simulink model "Buck"  (R2021b)
settings: Solver=VariableStepAuto  StartTime=0.0  StopTime=10.0  RelTol=1e-3
libraries: spsCurrentMeasurementLib x2, spsSeriesRLCBranchLib x2, spsDCVoltageSourceLib x1, spsDiodeLib x1, spsMosfetLib x1, spsVoltageMeasurementLib x1, spspowerguiLib x1
settings Model: Creator=szenia  LastModifiedBy=szenia

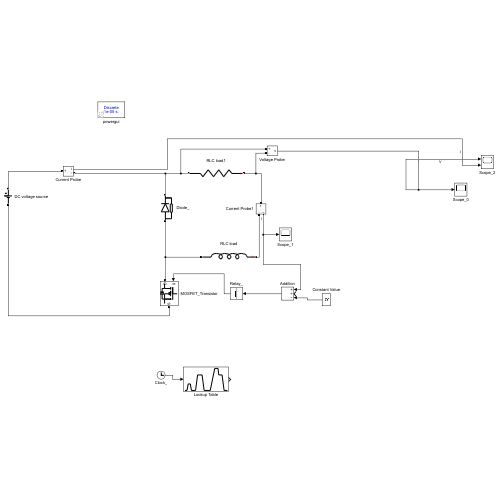
[thumbnail: Simulink's stored preview of the top-level diagram]
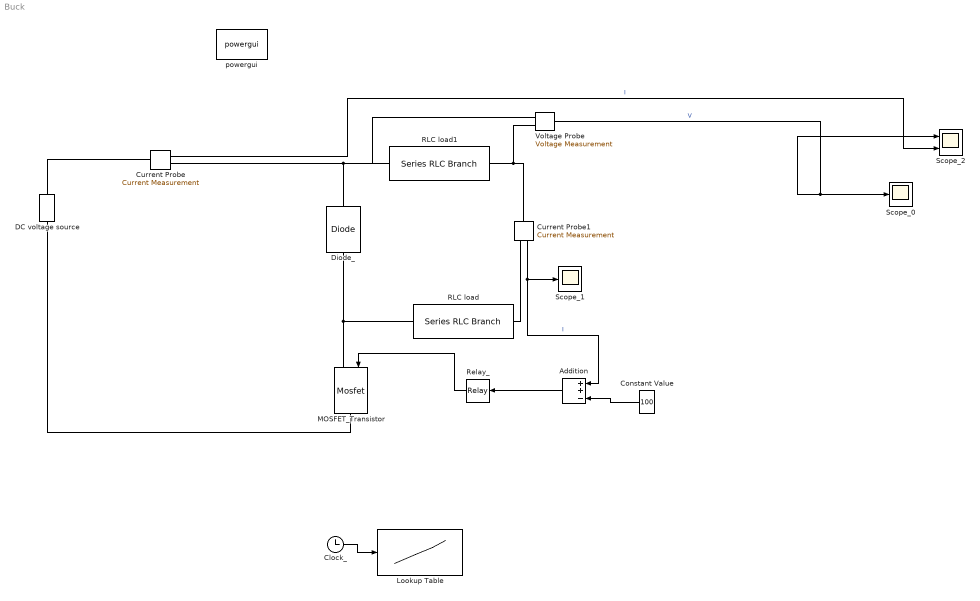
== system Buck ==
  Addition : Sum  Inputs=++-
  Clock_ : Clock
  Constant Value : Constant  Value=100
  Current Probe : spsCurrentMeasurementLib/Current Measurement  PhasorSimulation=off  OutputType=Complex  PSBequivalent=0
  Current Probe1 : spsCurrentMeasurementLib/Current Measurement  PhasorSimulation=off  OutputType=Complex  PSBequivalent=0
  DC voltage source : spsDCVoltageSourceLib/DC Voltage Source  Amplitude=250  Measurements=None
  Diode_ : spsDiodeLib/Diode  Ron=0.001  Lon=0  Vf=0.8  IC=0  UseSnubber=off  Rs=500  Cs=250e-9  Measurements=off
  Lookup Table : Lookup  InputValues=[0,10,15,25,30,50,60,80,90,120,140,155,160,175,185,200]  Table=[0,0,15,15,0,0,35,35,0,0,50,50,35,35,0,0]
  MOSFET_Transistor : spsMosfetLib/Mosfet  Ron=0.004  Lon=0  Rd=0.01  Vfd=0  IC=0  Rs=1e5  Cs=inf  Measurements=off
  RLC load : spsSeriesRLCBranchLib/Series RLC Branch  LConnTagsString=__new0  RConnTagsString=__new0  BranchType=L  Resistance=1  Inductance=10e-3  SetiL0=off  InitialCurrent=0  Capacitance=0  Setx0=off  InitialVoltage=0  Measurements=Branch current
  RLC load1 : spsSeriesRLCBranchLib/Series RLC Branch  LConnTagsString=__new0  RConnTagsString=__new0  BranchType=R  Resistance=1  Inductance=1e-2  SetiL0=off  InitialCurrent=0  Capacitance=0  Setx0=off  InitialVoltage=0  Measurements=Branch current
  Relay_ : Relay  OnSwitchValue=1  OffSwitchValue=-1  OnOutputValue=0  OffOutputValue=1
  Scope_0 : Scope
  Scope_1 : Scope
  Scope_2 : Scope  NumInputPorts=2
  Voltage Probe : spsVoltageMeasurementLib/Voltage Measurement  PhasorSimulation=off  OutputType=Complex  PSBequivalent=0
  powergui : spspowerguiLib/powergui  Priority=1  SimulationMode=Discrete  SampleTime=1e-5  frequency=60  Iterations=50  frequencyindice=0  Pbase=100e6  ErrMax=1e-4  UnitsV=kV  UnitsW=MW  buscounter=0  FunctionMessages=off  echomessages=off  EnableUseOfTLC=off  CurrentSourceSwitches=off  DisableSnubberDevices=off  DisableRonSwitches=off  DisableVfSwitches=off  DisplayEquations=off  AutomaticDiscreteSolvers=off  SolverType=Tustin/Backward Euler (TBE)  Interpol=off  ExternalGateDelay=off  methode=off  Ts=100  x0status=zero  SPID=on  SwTol=0  HookPort=off  NonlinearTolerance=1e-4  nMaxIteration=100  ContinueOnMaxIteration=off  RestoreLinks=warning  ResistiveCurrentMeasurement=off  Frange=[0:2:500]  Ylog=off  Xlog=on  ShowGrid=off  save=off  variable=ZData  structure=0  ZoomFFT=off  StartTime=0.0  cycles=1  DisplayStyle=1  fundamental=60  FreqAxis=off  MaxFrequency=1000  frequencyindicesteady=1  RmsSteady=1  display=off
  wires:
  Clock_/1 -> Lookup Table/1
  Current Probe/1 -> Scope_2/2  "I"
  Voltage Probe/1 -> Scope_2/1, Scope_0/1  "V"
  Current Probe1/1 -> Addition/1, Scope_1/1  "I"
  Relay_/1 -> MOSFET_Transistor/1
  Addition/1 -> Relay_/1
  Constant Value/1 -> Addition/3
  connections:
  Diode_/LConn1 -- RLC load/RConn1 -- MOSFET_Transistor/LConn1
  Diode_/RConn1 -- Voltage Probe/LConn1 -- RLC load1/RConn1 -- Current Probe/RConn1
  DC voltage source/RConn1 -- Current Probe/LConn1
  MOSFET_Transistor/RConn1 -- DC voltage source/LConn1
  Voltage Probe/LConn2 -- Current Probe1/LConn1 -- RLC load1/LConn1
  Current Probe1/RConn1 -- RLC load/LConn1
